simulink subsystem "HydrostaticCVT"  (R2025a)
settings: Solver=VariableStepAuto  StartTime=0.0  StopTime=10.0  RelTol=1e-3
undefined symbols (not defined in the file): fluids, hydrostaticCVT
libraries: fl_lib x48, nesl_utility x21, SimscapeFluids_lib x10
(part 1 of 2)
settings Model: Creator=varora  LastModifiedBy=varora

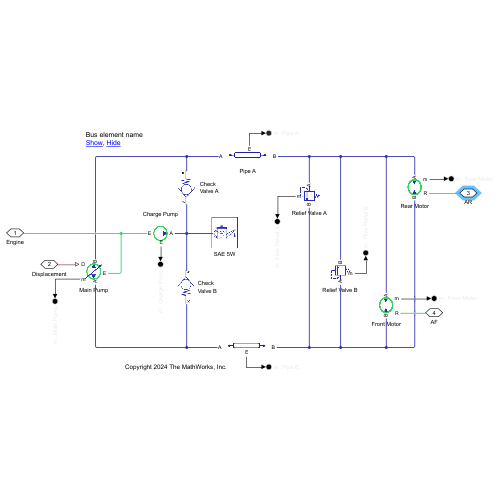
[thumbnail: Simulink's stored preview of the top-level diagram]
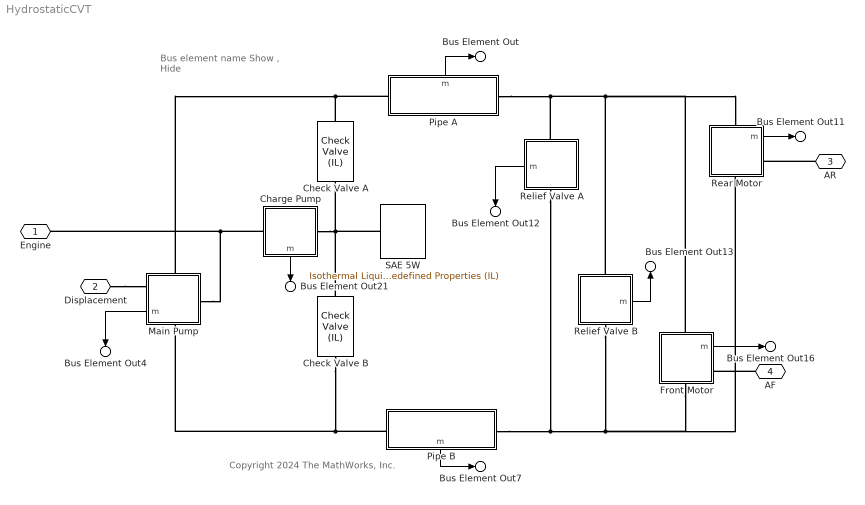
== system HydrostaticCVT ==
  note: Copyright 2024 The MathWorks, Inc.
  note: Bus element name
      | Show , Hide
  Charge Pump : Subsystem
      settings: PortSchema="{\"entries\":[{\"content\":{\"sides\":[{\"content\":{\"connectorIds\":[\"LConn1\"]},\"type\":\"ConnectorPlacement.EquallySpacedRectSide\",\"uuid\":\"81990219-23ac-4389-a887-166c20c53a41\"},{\"content\":{\"connectorIds\":[\"RConn1\"],\"side\":\"RIGHT\"},\"type\":\"ConnectorPlacement.EquallySpacedRectSide\",\"uuid\":\"3a415587-1da3-4934-b76c-e991c85e941a\"},{\"content\":{\"side\":\"TOP\"},\"type\":\"ConnectorPlacement.EquallySpacedRectSide\",\"uuid\":\"72b315a4-6c20-47a4-988f-efee67fcb81b\"},{\"content\":{\"connectorIds\":[\"Out1\"],\"side\":\"BOTTOM\"},\"type\":\"ConnectorPlacement.EquallySpacedRectSide\",\"uuid\":\"18a5ef52-f25e-4c35-ac51-885ef06c2aba\"}]},\"type\":\"ConnectorPlacement.EquallySpacedConnector\",\"uuid\":\"73b5088a-800b-40b1-b457-59a8e6f658c4\"}],\"packageUris\":[\"http://schema.mathworks.com/mf0/Connector/R2020b\"],\"version\":\"1.0\"}"
      mask Display: image('Fixed Displacement Pump.png');
  Check Valve A : SimscapeFluids_lib/Isothermal Liquid/Valves & Orifices/Directional Control Valves/Check Valve (IL)  opening_spec=2*(fluids.isothermal_liquid.valves_orifices.enum.PressureOpeningSpec.Linear)-1  pressure_control_spec=fluids.isothermal_liquid.valves_orifices.enum.pressure_control_spec.dp  p_crack_differential=hydrostaticCVT.pressDifferentialCracking MPa  p_crack_gauge=0.1 MPa  press_max_differential="hydrostaticCVT.pressDifferentialMaxOpen   MPa"  press_max_gauge=0.2 MPa  area_max=hydrostaticCVT.areaMax m^2  area_leak=hydrostaticCVT.areaLeak m^2  p_diff_TLU=[0.01 : 0.01 : 0.1] MPa  valve_area_TLU=[1e-10, 1e-05, 2e-05, 3e-05, 4e-05, 5e-05, 6e-05, 7.5e-05, 8.5e-05, .0001] m^2  vol_flow_TLU=[.000358, .045, .11, .191, .284, .39, .505, .63, .764, .905] .* 1e-3 m^3/s  area=inf m^2  Cd=hydrostaticCVT.cd  Re_c=150  smoothing_factor=0.01  pressure_recovery=simscape.enum.onoff.off  opening_dynamics=simscape.enum.onoff.off  tau=0.1 s
      settings: InternalSimscapePortConfiguration="{\"Bottom\":[],\"Left\":[{\"id\":\"A\",\"label\":\"A\",\"type\":\"foundation.isothermal_liquid.isothermal_liquid\"}],\"Right\":[{\"id\":\"B\",\"label\":\"B\",\"type\":\"foundation.isothermal_liquid.isothermal_liquid\"}],\"Top\":[]}"
  Check Valve B : SimscapeFluids_lib/Isothermal Liquid/Valves & Orifices/Directional Control Valves/Check Valve (IL)  opening_spec=2*(fluids.isothermal_liquid.valves_orifices.enum.PressureOpeningSpec.Linear)-1  pressure_control_spec=fluids.isothermal_liquid.valves_orifices.enum.pressure_control_spec.dp  p_crack_differential=hydrostaticCVT.pressDifferentialCracking MPa  p_crack_gauge=0.1 MPa  press_max_differential="hydrostaticCVT.pressDifferentialMaxOpen   MPa"  press_max_gauge=0.2 MPa  area_max=hydrostaticCVT.areaMax m^2  area_leak=hydrostaticCVT.areaLeak m^2  p_diff_TLU=[0.01 : 0.01 : 0.1] MPa  valve_area_TLU=[1e-10, 1e-05, 2e-05, 3e-05, 4e-05, 5e-05, 6e-05, 7.5e-05, 8.5e-05, .0001] m^2  vol_flow_TLU=[.000358, .045, .11, .191, .284, .39, .505, .63, .764, .905] .* 1e-3 m^3/s  area=inf m^2  Cd=hydrostaticCVT.cd  Re_c=150  smoothing_factor=0.01  pressure_recovery=simscape.enum.onoff.off  opening_dynamics=simscape.enum.onoff.off  tau=0.1 s
      settings: InternalSimscapePortConfiguration="{\"Bottom\":[],\"Left\":[{\"id\":\"A\",\"label\":\"A\",\"type\":\"foundation.isothermal_liquid.isothermal_liquid\"}],\"Right\":[{\"id\":\"B\",\"label\":\"B\",\"type\":\"foundation.isothermal_liquid.isothermal_liquid\"}],\"Top\":[]}"
  Front Motor : Subsystem
      settings: PortSchema="{\"entries\":[{\"content\":{\"sides\":[{\"content\":{},\"type\":\"ConnectorPlacement.EquallySpacedRectSide\",\"uuid\":\"af94f2aa-b04e-40af-a187-0818155794dd\"},{\"content\":{\"connectorIds\":[\"Out1\",\"RConn1\"],\"side\":\"RIGHT\"},\"type\":\"ConnectorPlacement.EquallySpacedRectSide\",\"uuid\":\"5c20c2e1-8527-47fe-9ffe-16d60e314a5b\"},{\"content\":{\"connectorIds\":[\"LConn1\"],\"side\":\"TOP\"},\"type\":\"ConnectorPlacement.EquallySpacedRectSide\",\"uuid\":\"e7f5e70d-3df0-46cd-83a4-29ec656a12c9\"},{\"content\":{\"connectorIds\":[\"RConn2\"],\"side\":\"BOTTOM\"},\"type\":\"ConnectorPlacement.EquallySpacedRectSide\",\"uuid\":\"f2252cf3-f3a6-42d9-8396-2baa411525c5\"}]},\"type\":\"ConnectorPlacement.EquallySpacedConnector\",\"uuid\":\"0c7ba87d-5f8c-4429-8766-c6dc02a36f7b\"}],\"packageUris\":[\"http://schema.mathworks.com/mf0/Connector/R2020b\"],\"version\":\"1.0\"}"
      mask Display: image('Fixed Displacement Motor.png');
  Main Pump : Subsystem
      settings: PortSchema="{\"entries\":[{\"content\":{\"sides\":[{\"content\":{\"connectorIds\":[\"LConn1\",\"Out1\"]},\"type\":\"ConnectorPlacement.EquallySpacedRectSide\",\"uuid\":\"857969f3-473a-4560-b879-851e5f4c83b0\"},{\"content\":{\"connectorIds\":[\"RConn1\"],\"side\":\"RIGHT\"},\"type\":\"ConnectorPlacement.EquallySpacedRectSide\",\"uuid\":\"4f69d4a9-a494-47de-b36f-c1227f8f36db\"},{\"content\":{\"connectorIds\":[\"LConn2\"],\"side\":\"TOP\"},\"type\":\"ConnectorPlacement.EquallySpacedRectSide\",\"uuid\":\"5719fdc2-cb8a-4698-a7b4-0c22c79051ee\"},{\"content\":{\"connectorIds\":[\"RConn2\"],\"side\":\"BOTTOM\"},\"type\":\"ConnectorPlacement.EquallySpacedRectSide\",\"uuid\":\"9c51d1b2-abf1-46a3-9cf9-9060aeca44d8\"}]},\"type\":\"ConnectorPlacement.EquallySpacedConnector\",\"uuid\":\"aaa09012-c93e-45df-8a88-38540d88c81c\"}],\"packageUris\":[\"http://schema.mathworks.com/mf0/Connector/R2020b\"],\"version\":\"1.0\"}"
      mask Display: image('Variable Displacement Pump.png');
  Pipe A : Subsystem
      settings: PortSchema="{\"entries\":[{\"content\":{\"sides\":[{\"content\":{\"connectorIds\":[\"LConn1\"]},\"type\":\"ConnectorPlacement.EquallySpacedRectSide\",\"uuid\":\"d71b6971-6f33-4ff5-9472-1e7ceb29be5c\"},{\"content\":{\"connectorIds\":[\"RConn1\"],\"side\":\"RIGHT\"},\"type\":\"ConnectorPlacement.EquallySpacedRectSide\",\"uuid\":\"20efd35b-04f1-44a0-a5ae-b6ecc8cce91a\"},{\"content\":{\"connectorIds\":[\"Out1\"],\"side\":\"TOP\"},\"type\":\"ConnectorPlacement.EquallySpacedRectSide\",\"uuid\":\"941ffbf3-e51b-4589-ab00-835957186b5f\"}]},\"type\":\"ConnectorPlacement.EquallySpacedConnector\",\"uuid\":\"7b30b026-434b-4245-94a4-5fd456974538\"}],\"packageUris\":[\"http://schema.mathworks.com/mf0/Connector/R2020b\"],\"version\":\"1.0\"}"
      mask Display: image('Pipe.png');
  Pipe B : Subsystem
      settings: PortSchema="{\"entries\":[{\"content\":{\"sides\":[{\"content\":{\"connectorIds\":[\"LConn1\"]},\"type\":\"ConnectorPlacement.EquallySpacedRectSide\",\"uuid\":\"d71b6971-6f33-4ff5-9472-1e7ceb29be5c\"},{\"content\":{\"connectorIds\":[\"RConn1\"],\"side\":\"RIGHT\"},\"type\":\"ConnectorPlacement.EquallySpacedRectSide\",\"uuid\":\"20efd35b-04f1-44a0-a5ae-b6ecc8cce91a\"},{\"content\":{\"side\":\"TOP\"},\"type\":\"ConnectorPlacement.EquallySpacedRectSide\",\"uuid\":\"941ffbf3-e51b-4589-ab00-835957186b5f\"},{\"content\":{\"connectorIds\":[\"Out1\"],\"side\":\"BOTTOM\"},\"type\":\"ConnectorPlacement.EquallySpacedRectSide\",\"uuid\":\"a318eed9-4e9d-48d8-b72b-a2a7d74f41ab\"}]},\"type\":\"ConnectorPlacement.EquallySpacedConnector\",\"uuid\":\"7b30b026-434b-4245-94a4-5fd456974538\"}],\"packageUris\":[\"http://schema.mathworks.com/mf0/Connector/R2020b\"],\"version\":\"1.0\"}"
      mask Display: image('Pipe.png');
  Rear Motor : Subsystem
      settings: PortSchema="{\"entries\":[{\"content\":{\"sides\":[{\"content\":{},\"type\":\"ConnectorPlacement.EquallySpacedRectSide\",\"uuid\":\"af94f2aa-b04e-40af-a187-0818155794dd\"},{\"content\":{\"connectorIds\":[\"Out1\",\"RConn1\"],\"side\":\"RIGHT\"},\"type\":\"ConnectorPlacement.EquallySpacedRectSide\",\"uuid\":\"5c20c2e1-8527-47fe-9ffe-16d60e314a5b\"},{\"content\":{\"connectorIds\":[\"LConn1\"],\"side\":\"TOP\"},\"type\":\"ConnectorPlacement.EquallySpacedRectSide\",\"uuid\":\"e7f5e70d-3df0-46cd-83a4-29ec656a12c9\"},{\"content\":{\"connectorIds\":[\"RConn2\"],\"side\":\"BOTTOM\"},\"type\":\"ConnectorPlacement.EquallySpacedRectSide\",\"uuid\":\"960debcf-3e01-48e5-86cf-b4bb7f8de203\"}]},\"type\":\"ConnectorPlacement.EquallySpacedConnector\",\"uuid\":\"0c7ba87d-5f8c-4429-8766-c6dc02a36f7b\"}],\"packageUris\":[\"http://schema.mathworks.com/mf0/Connector/R2020b\"],\"version\":\"1.0\"}"
      mask Display: image('Fixed Displacement Motor.png');
  Relief Valve A : Subsystem
      settings: PortSchema="{\"entries\":[{\"content\":{\"sides\":[{\"content\":{\"connectorIds\":[\"LConn1\"]},\"type\":\"ConnectorPlacement.EquallySpacedRectSide\",\"uuid\":\"a381c46d-7477-4f99-8d1a-7d1a868f6356\"},{\"content\":{\"connectorIds\":[\"RConn1\"],\"side\":\"RIGHT\"},\"type\":\"ConnectorPlacement.EquallySpacedRectSide\",\"uuid\":\"1773284f-5c53-4cb3-9146-19bcc89e0bf2\"},{\"content\":{\"connectorIds\":[\"Out1\"],\"side\":\"TOP\"},\"type\":\"ConnectorPlacement.EquallySpacedRectSide\",\"uuid\":\"2cc97cf0-3f11-430a-9e32-d4b384bcc7e2\"}]},\"type\":\"ConnectorPlacement.EquallySpacedConnector\",\"uuid\":\"a3df120c-9f95-4600-8cbc-77d57dad487f\"}],\"packageUris\":[\"http://schema.mathworks.com/mf0/Connector/R2020b\"],\"version\":\"1.0\"}"
      mask Display: image('Relief Valve.png');
  Relief Valve B : Subsystem
      settings: PortSchema="{\"entries\":[{\"content\":{\"sides\":[{\"content\":{\"connectorIds\":[\"LConn1\"]},\"type\":\"ConnectorPlacement.EquallySpacedRectSide\",\"uuid\":\"a381c46d-7477-4f99-8d1a-7d1a868f6356\"},{\"content\":{\"connectorIds\":[\"RConn1\"],\"side\":\"RIGHT\"},\"type\":\"ConnectorPlacement.EquallySpacedRectSide\",\"uuid\":\"1773284f-5c53-4cb3-9146-19bcc89e0bf2\"},{\"content\":{\"side\":\"TOP\"},\"type\":\"ConnectorPlacement.EquallySpacedRectSide\",\"uuid\":\"2cc97cf0-3f11-430a-9e32-d4b384bcc7e2\"},{\"content\":{\"connectorIds\":[\"Out1\"],\"side\":\"BOTTOM\"},\"type\":\"ConnectorPlacement.EquallySpacedRectSide\",\"uuid\":\"486595bc-126c-4ff1-8e4a-4a4a030a425b\"}]},\"type\":\"ConnectorPlacement.EquallySpacedConnector\",\"uuid\":\"a3df120c-9f95-4600-8cbc-77d57dad487f\"}],\"packageUris\":[\"http://schema.mathworks.com/mf0/Connector/R2020b\"],\"version\":\"1.0\"}"
      mask Display: image('Relief Valve.png');
  SAE 5W : SimscapeFluids_lib/Isothermal Liquid/Utilities/Isothermal Liquid Predefined Properties (IL)  fluid_list=fluids.isothermal_liquid.utilities.enum.isothermal_liquid_fluid_list.sae5w30  concentration_param_EG=fluids.isothermal_liquid.utilities.enum.isothermal_liquid_concentration.volume_fraction  concentration_param_PG=fluids.isothermal_liquid.utilities.enum.isothermal_liquid_concentration.volume_fraction  c_mass_SW=3.5e-3  c_mass_EG=0.1  c_mass_PG=0.1  c_mass_GL=0.1  c_vol_EG=0.1  c_vol_PG=0.1  beta_L_atm_EG=2.1791 GPa  beta_L_atm_PG=2.1791 GPa  beta_L_atm_GL=2.1791 GPa  p_min_EG=0.01 MPa  p_min_PG=0.01 MPa  p_min_GL=0.01 MPa  T=293.15 K  derate_coeff=1  p_atm=0.101325 MPa  properties_range_check=simscape.enum.assert.action.error  air_fraction=0.02  polytropic_index=1.0  rho_g_atm=1.225 kg/m^3  air_dissolution_model=simscape.enum.onoff.off  p_crit=3 MPa
      settings: InternalSimscapePortConfiguration="{\"Bottom\":[],\"Left\":[],\"Right\":[{\"id\":\"A\",\"label\":\"\",\"type\":\"foundation.isothermal_liquid.isothermal_liquid\"}],\"Top\":[]}"
  Engine : PMIOPort  Side=Left
  Displacement : PMIOPort  Port=2  Side=Left
  AR : PMIOPort  Port=3  Side=Right
  AF : PMIOPort  Port=4  Side=Right
  Bus Element Out : Outport  PortName=m  Element=Pipe A
  Bus Element Out4 : Outport  PortName=m  Element=Main Pump
  Bus Element Out7 : Outport  PortName=m  Element=Pipe B
  Bus Element Out11 : Outport  PortName=m  Element=Rear Motor
  Bus Element Out12 : Outport  PortName=m  Element=Flow Relief A
  Bus Element Out13 : Outport  PortName=m  Element=Flow Relief B
  Bus Element Out16 : Outport  PortName=m  Element=Front Motor
  Bus Element Out21 : Outport  PortName=m  Element=Charge Pump
  wires:
  Main Pump/1(m) -> Bus Element Out4/1
  Pipe A/1(m) -> Bus Element Out/1
  Pipe B/1(m) -> Bus Element Out7/1
  Front Motor/1(m) -> Bus Element Out16/1
  Rear Motor/1(m) -> Bus Element Out11/1
  Relief Valve A/1(m) -> Bus Element Out12/1
  Relief Valve B/1(m) -> Bus Element Out13/1
  Charge Pump/1(m) -> Bus Element Out21/1
  connections:
  Main Pump/LConn2 -- Pipe A/LConn1 -- Check Valve A/RConn1
  SAE 5W/RConn1 -- Charge Pump/RConn1 -- Check Valve B/LConn1 -- Check Valve A/LConn1
  Pipe A/RConn1 -- Rear Motor/LConn1 -- Front Motor/LConn1 -- Relief Valve B/RConn1 -- Relief Valve A/LConn1
  Pipe B/LConn1 -- Check Valve B/RConn1 -- Main Pump/RConn2
  Pipe B/RConn1 -- Rear Motor/RConn2 -- Front Motor/RConn2 -- Relief Valve B/LConn1 -- Relief Valve A/RConn1
  Main Pump/RConn1 -- Charge Pump/LConn1 -- Engine/RConn1
  Displacement/RConn1 -- Main Pump/LConn1
  AF/RConn1 -- Front Motor/RConn1
  AR/RConn1 -- Rear Motor/RConn1

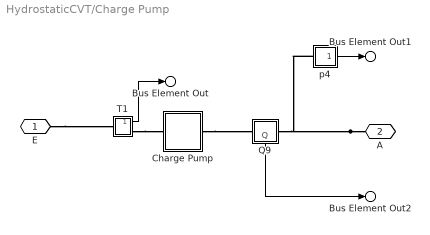
== system HydrostaticCVT/Charge Pump ==
  Charge Pump : Subsystem  Tag=PublishSubsystem
      mask Display:
      | % Circle
      | plot(2*cos(linspace(0, 2*pi, 100)), 2*sin(linspace(0, 2*pi, 100)))
      | % Triangle
      | patch([1 0.4 0.4]*2, [0,-0.4,0.4]*2)
      | % Boundary
      | color('white')
      | plot(-2, -2)
      | plot(2, 2)
  Q9 : Subsystem
      settings: PortSchema="{\"entries\":[{\"content\":{\"sides\":[{\"content\":{},\"type\":\"ConnectorPlacement.EquallySpacedRectSide\",\"uuid\":\"a381c46d-7477-4f99-8d1a-7d1a868f6356\"},{\"content\":{\"connectorIds\":[\"Out1\"],\"side\":\"RIGHT\"},\"type\":\"ConnectorPlacement.EquallySpacedRectSide\",\"uuid\":\"1773284f-5c53-4cb3-9146-19bcc89e0bf2\"},{\"content\":{\"connectorIds\":[\"LConn1\"],\"side\":\"TOP\"},\"type\":\"ConnectorPlacement.EquallySpacedRectSide\",\"uuid\":\"2cc97cf0-3f11-430a-9e32-d4b384bcc7e2\"},{\"content\":{\"connectorIds\":[\"RConn1\"],\"side\":\"BOTTOM\"},\"type\":\"ConnectorPlacement.EquallySpacedRectSide\",\"uuid\":\"6b1044f7-a51c-47fb-9697-f1e3b42da025\"}]},\"type\":\"ConnectorPlacement.EquallySpacedConnector\",\"uuid\":\"a3df120c-9f95-4600-8cbc-77d57dad487f\"}],\"packageUris\":[\"http://schema.mathworks.com/mf0/Connector/R2020b\"],\"version\":\"1.0\"}"
      mask Display: disp('Q')
  T1 : Subsystem
      mask Display: disp('S')
  p4 : Subsystem
      mask Display: disp('P')
  E : PMIOPort  Side=Left
  A : PMIOPort  Port=2  Side=Right
  Bus Element Out : Outport  PortName=m  Element=trq (N*m)
  Bus Element Out1 : Outport  PortName=m  Element=P (bar)
  Bus Element Out2 : Outport  PortName=m  Element=q (m^3/s)
  wires:
  Q9/1(Q) -> Bus Element Out2/1
  p4/1(" P") -> Bus Element Out1/1
  T1/1(T) -> Bus Element Out/1
  connections:
  T1/RConn1 -- Charge Pump/LConn1
  Charge Pump/RConn1 -- Q9/RConn1
  E/RConn1 -- T1/LConn1
  A/RConn1 -- Q9/LConn1 -- p4/LConn1

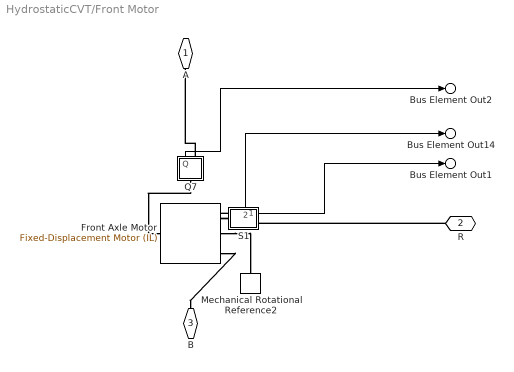
== system HydrostaticCVT/Front Motor ==
  Front Axle Motor : SimscapeFluids_lib/Isothermal Liquid/Pumps & Motors/Fixed-Displacement Motor (IL)  leakage_friction_spec=fluids.isothermal_liquid.pumps_motors.enum.MotorLossSpec.Analytical  displacement=hydrostaticCVT.displacementMotor cm^3/rev  omega_nominal=hydrostaticCVT.shaftVelocityNominal rpm  p_nominal=hydrostaticCVT.nominalPressureGain MPa  vol_eff_nominal=hydrostaticCVT.efficiencyVolumetric  mech_eff_nominal=hydrostaticCVT.efficiencyMechanical  no_load_torque=0 N*m  p_diff_eff_TLU=[.1, 1, 2] MPa  omega_eff_TLU=[25, 50, 100, 200, 300, 400] rad/s  vol_eff_TLU=[.816, .908, .954, .977, .981, .984; .325, .663, .831, .916, .925, .946; .137, .568, .78, .892, .893, .91]  mech_eff_TLU=[.996, .996, .996, .996, .996, .996; .988, .989, .989, .989, .989, .99; .981, .981, .982, .982, .983, .984]  p_diff_loss_TLU=[.1, 1, 2] MPa  omega_loss_TLU=[25, 50, 100, 200, 300, 400] rad/s  vol_loss_TLU=[.023, .023, .023, .023, .0285, .032; .0844, .0842, .0845, .084, .1125, .108; .1079, .108, .11, .108, .1605, .18] * 1e-3 m^3/s  mech_loss_TLU=[.002, .002, .002, .002, .002, .002; .0607, .0556, .0556, .0556, .0556, .0505; .1937, .1937, .1833, .1833, .1729, .1626] N*m  q_shaft_TLU=[.125, .25, .5, 1, 1.5, 2] * 1e-3 m^3/s  p_diff_shaft_TLU=[.1, 1, 2] MPa  torque_shaft_TLU=[.47, 4.72, 9.35; .47, 4.7, 9.36; .47, 4.7, 9.4; .47, 4.7, 9.41; .47, 4.7, 9.46; .47, 4.68, 9.5] N*m  omega_shaft_TLU=[205, 80, 35; 455, 330, 285; 955, 831, 780; 1950, 1830, 1780; 2940, 2775, 2680; 3940, 3780, 3640] rpm  vol_eff_min=1e-3  vol_eff_max=1  mech_eff_min=1e-3  mech_eff_max=1  pressure_threshold=1e-3 MPa  omega_threshold=10 rad/s  supplied_range_check=simscape.enum.assert.action.none  motor_mode_check=simscape.enum.assert.action.none  pressure_check=simscape.enum.assert.action.none  p_min_valid=0.101325 MPa
      settings: InternalSimscapePortConfiguration="{\"Bottom\":[{\"id\":\"B\",\"label\":\"B\",\"type\":\"foundation.isothermal_liquid.isothermal_liquid\"}],\"Left\":[],\"Right\":[{\"id\":\"R\",\"label\":\"R\",\"type\":\"foundation.mechanical.rotational.rotational\"},{\"id\":\"C\",\"label\":\"C\",\"type\":\"foundation.mechanical.rotational.rotational\"}],\"Top\":[{\"id\":\"A\",\"label\":\"A\",\"type\":\"foundation.isothermal_liquid.isothermal_liquid\"}]}"
  Mechanical Rotational Reference2 : fl_lib/Mechanical/Rotational Elements/Mechanical Rotational Reference
  Q7 : Subsystem
      mask Display: disp('Q')
  S1 : Subsystem
      settings: PortSchema="{\"entries\":[{\"content\":{\"sides\":[{\"content\":{\"connectorIds\":[\"LConn1\"]},\"type\":\"ConnectorPlacement.EquallySpacedRectSide\",\"uuid\":\"d71b6971-6f33-4ff5-9472-1e7ceb29be5c\"},{\"content\":{\"connectorIds\":[\"Out1\",\"RConn1\"],\"side\":\"RIGHT\"},\"type\":\"ConnectorPlacement.EquallySpacedRectSide\",\"uuid\":\"20efd35b-04f1-44a0-a5ae-b6ecc8cce91a\"},{\"content\":{\"connectorIds\":[\"Out2\"],\"side\":\"TOP\"},\"type\":\"ConnectorPlacement.EquallySpacedRectSide\",\"uuid\":\"941ffbf3-e51b-4589-ab00-835957186b5f\"}]},\"type\":\"ConnectorPlacement.EquallySpacedConnector\",\"uuid\":\"7b30b026-434b-4245-94a4-5fd456974538\"}],\"packageUris\":[\"http://schema.mathworks.com/mf0/Connector/R2020b\"],\"version\":\"1.0\"}"
      mask Display: disp('S')
  A : PMIOPort  Side=Left
  R : PMIOPort  Port=2  Side=Right
  B : PMIOPort  Port=3  Side=Right
  Bus Element Out14 : Outport  PortName=m  Element=w (rpm)
  Bus Element Out1 : Outport  PortName=m  Element=trq (N*m)
  Bus Element Out2 : Outport  PortName=m  Element=q (m^3/s)
  wires:
  Q7/1(Q) -> Bus Element Out2/1
  S1/1(T (N*m)) -> Bus Element Out1/1
  S1/2(w (rpm)) -> Bus Element Out14/1
  connections:
  Q7/RConn1 -- A/RConn1
  Front Axle Motor/RConn3 -- B/RConn1
  Front Axle Motor/RConn2 -- Mechanical Rotational Reference2/LConn1
  R/RConn1 -- S1/RConn1
  Q7/LConn1 -- Front Axle Motor/LConn1
  S1/LConn1 -- Front Axle Motor/RConn1

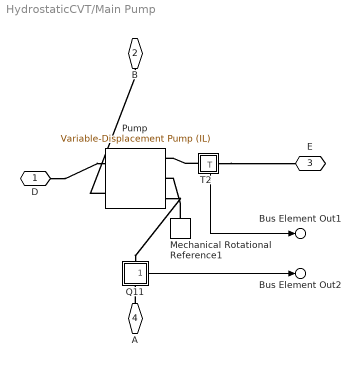
== system HydrostaticCVT/Main Pump ==
  Mechanical Rotational Reference1 : fl_lib/Mechanical/Rotational Elements/Mechanical Rotational Reference
  Pump : SimscapeFluids_lib/Isothermal Liquid/Pumps & Motors/Variable-Displacement Pump (IL)  leakage_friction_spec=fluids.isothermal_liquid.pumps_motors.enum.pump_motor_loss_spec.analytical  displacement_nominal=hydrostaticCVT.displacementPump cm^3/rev  omega_nominal=hydrostaticCVT.shaftVelocityNominal rpm  p_nominal=hydrostaticCVT.nominalPressureGain MPa  vol_eff_nominal=hydrostaticCVT.efficiencyVolumetric  mech_eff_nominal=hydrostaticCVT.efficiencyMechanical  no_load_torque=0 N*m  p_diff_eff_TLU=[.1, 1, 2] MPa  omega_eff_TLU=[25, 50, 100, 200, 300, 400] rad/s  displacement_eff_TLU=[-30, -19, 19, 30] cm^3/rev  vol_eff_TLU=repmat([.816, .908, .954, .977, .981, .984; .325, .663, .831, .916, .925, .946; .137, .568, .78, .892, .893, .91], 1, 1, 4)  mech_eff_TLU=repmat([.996, .996, .996, .996, .996, .996; .988, .989, .989, .989, .989, .99; .981, .981, .982, .982, .983, .984], 1, 1, 4)  p_diff_loss_TLU=[.1, 1, 2] MPa  omega_loss_TLU=[25, 50, 100, 200, 300, 400] rad/s  displacement_loss_TLU=[-30, -19, 19, 30] cm^3/rev  vol_loss_TLU=repmat([.023, .023, .023, .023, .0285, .032; .0844, .0842, .0845, .084, .1125, .108; .1079, .108, .11, .108, .1605, .18] * 1e-3, 1, 1, 4) m^3/s  mech_loss_TLU=repmat([.002, .002, .002, .002, .002, .002; .0607, .0556, .0556, .0556, .0556, .0505; .1937, .1937, .1833, .1833, .1729, .1626], 1, 1, 4) N*m  vol_eff_min=1e-3  vol_eff_max=1  mech_eff_min=1e-3  mech_eff_max=1  pressure_threshold=1e-3 MPa  omega_threshold=10 rad/s  displacement_threshold=0.1 cm^3/rev  supplied_range_check=simscape.enum.assert.action.none  pump_mode_check=simscape.enum.assert.action.none  pressure_check=simscape.enum.assert.action.none  p_min_valid=0.101325 MPa
      settings: InternalSimscapePortConfiguration="{\"Bottom\":[{\"id\":\"A\",\"label\":\"A\",\"type\":\"foundation.isothermal_liquid.isothermal_liquid\"}],\"Left\":[{\"id\":\"D\",\"label\":\"D\",\"type\":\"input\"}],\"Right\":[{\"id\":\"R\",\"label\":\"R\",\"type\":\"foundation.mechanical.rotational.rotational\"},{\"id\":\"C\",\"label\":\"C\",\"type\":\"foundation.mechanical.rotational.rotational\"}],\"Top\":[{\"id\":\"B\",\"label\":\"B\",\"type\":\"foundation.isothermal_liquid.isothermal_liquid\"}]}"
  Q11 : Subsystem
      settings: PortSchema="{\"entries\":[{\"content\":{\"sides\":[{\"content\":{\"connectorIds\":[\"LConn1\"]},\"type\":\"ConnectorPlacement.EquallySpacedRectSide\",\"uuid\":\"a381c46d-7477-4f99-8d1a-7d1a868f6356\"},{\"content\":{\"connectorIds\":[\"RConn1\"],\"side\":\"RIGHT\"},\"type\":\"ConnectorPlacement.EquallySpacedRectSide\",\"uuid\":\"1773284f-5c53-4cb3-9146-19bcc89e0bf2\"},{\"content\":{\"side\":\"TOP\"},\"type\":\"ConnectorPlacement.EquallySpacedRectSide\",\"uuid\":\"2cc97cf0-3f11-430a-9e32-d4b384bcc7e2\"},{\"content\":{\"connectorIds\":[\"Out1\"],\"side\":\"BOTTOM\"},\"type\":\"ConnectorPlacement.EquallySpacedRectSide\",\"uuid\":\"73fb13f1-32e6-4f88-8a39-50ddc70c8cb7\"}]},\"type\":\"ConnectorPlacement.EquallySpacedConnector\",\"uuid\":\"a3df120c-9f95-4600-8cbc-77d57dad487f\"}],\"packageUris\":[\"http://schema.mathworks.com/mf0/Connector/R2020b\"],\"version\":\"1.0\"}"
      mask Display: disp('Q')
  T2 : Subsystem
      settings: PortSchema="{\"entries\":[{\"content\":{\"sides\":[{\"content\":{\"connectorIds\":[\"LConn1\"]},\"type\":\"ConnectorPlacement.EquallySpacedRectSide\",\"uuid\":\"a381c46d-7477-4f99-8d1a-7d1a868f6356\"},{\"content\":{\"connectorIds\":[\"RConn1\"],\"side\":\"RIGHT\"},\"type\":\"ConnectorPlacement.EquallySpacedRectSide\",\"uuid\":\"1773284f-5c53-4cb3-9146-19bcc89e0bf2\"},{\"content\":{\"side\":\"TOP\"},\"type\":\"ConnectorPlacement.EquallySpacedRectSide\",\"uuid\":\"2cc97cf0-3f11-430a-9e32-d4b384bcc7e2\"},{\"content\":{\"connectorIds\":[\"Out1\"],\"side\":\"BOTTOM\"},\"type\":\"ConnectorPlacement.EquallySpacedRectSide\",\"uuid\":\"68438fb6-2ad6-4198-8251-4c01567bf9f2\"}]},\"type\":\"ConnectorPlacement.EquallySpacedConnector\",\"uuid\":\"a3df120c-9f95-4600-8cbc-77d57dad487f\"}],\"packageUris\":[\"http://schema.mathworks.com/mf0/Connector/R2020b\"],\"version\":\"1.0\"}"
      mask Display: disp('S')
  D : PMIOPort  Side=Left
  B : PMIOPort  Port=2  Side=Left
  E : PMIOPort  Port=3  Side=Right
  A : PMIOPort  Port=4  Side=Right
  Bus Element Out1 : Outport  PortName=m  Element=trq (N*m)
  Bus Element Out2 : Outport  PortName=m  Element=q (m^3/s)
  wires:
  Q11/1(Q) -> Bus Element Out2/1
  T2/1(T) -> Bus Element Out1/1
  connections:
  A/RConn1 -- Q11/LConn1
  Pump/RConn3 -- Q11/RConn1
  Pump/LConn2 -- B/RConn1
  D/RConn1 -- Pump/LConn1
  T2/LConn1 -- E/RConn1
  Mechanical Rotational Reference1/LConn1 -- Pump/RConn2
  T2/RConn1 -- Pump/RConn1

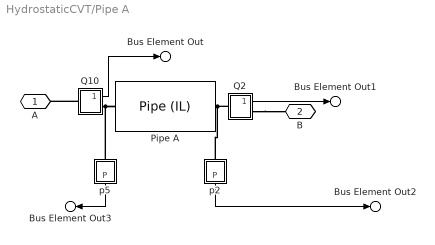
== system HydrostaticCVT/Pipe A ==
  Pipe A : fl_lib/Isothermal Liquid/Elements/Pipe (IL)  length=hydrostaticCVT.lengthPipe m  area=pi * hydrostaticCVT.diameterPipe^2 / 4 m^2  Dh=hydrostaticCVT.diameterPipe m  length_add=hydrostaticCVT.lengthPipe*0.5 m  roughness=30e-6 m  Re_lam=2000  Re_tur=4000  shape_factor=64  dynamic_compressibility=simscape.enum.onoff.on  inertia=simscape.enum.onoff.off  p0=0.101325 MPa  mdot0=0 kg/s
      settings: InternalSimscapePortConfiguration="{\"Bottom\":[],\"Left\":[{\"id\":\"A\",\"label\":\"A\",\"type\":\"foundation.isothermal_liquid.isothermal_liquid\"}],\"Right\":[{\"id\":\"B\",\"label\":\"B\",\"type\":\"foundation.isothermal_liquid.isothermal_liquid\"}],\"Top\":[]}"
  Q10 : Subsystem
      mask Display: disp('Q')
  Q2 : Subsystem
      mask Display: disp('Q')
  p2 : Subsystem
      mask Display: disp('P')
  p5 : Subsystem
      mask Display: disp('P')
  A : PMIOPort  Side=Left
  B : PMIOPort  Port=2  Side=Right
  Bus Element Out : Outport  PortName=m  Element=qA (m^3/s)
  Bus Element Out1 : Outport  PortName=m  Element=qB (m^3/s)
  Bus Element Out2 : Outport  PortName=m  Element=pB (bar)
  Bus Element Out3 : Outport  PortName=m  Element=pA (bar)
  wires:
  p5/1(" P") -> Bus Element Out3/1
  p2/1(" P") -> Bus Element Out2/1
  Q2/1(Q) -> Bus Element Out1/1
  Q10/1(Q) -> Bus Element Out/1
  connections:
  Q2/RConn1 -- B/RConn1
  Q10/LConn1 -- A/RConn1
  p2/LConn1 -- Q2/LConn1 -- Pipe A/RConn1
  p5/LConn1 -- Pipe A/LConn1 -- Q10/RConn1

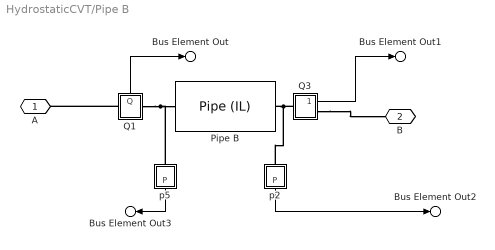
== system HydrostaticCVT/Pipe B ==
  Pipe B : fl_lib/Isothermal Liquid/Elements/Pipe (IL)  length=hydrostaticCVT.lengthPipe m  area=pi * hydrostaticCVT.diameterPipe^2 / 4 m^2  Dh=hydrostaticCVT.diameterPipe m  length_add=hydrostaticCVT.lengthPipe*0.5 m  roughness=30e-6 m  Re_lam=2000  Re_tur=4000  shape_factor=64  dynamic_compressibility=simscape.enum.onoff.on  inertia=simscape.enum.onoff.off  p0=0.101325 MPa  mdot0=0 kg/s
      settings: InternalSimscapePortConfiguration="{\"Bottom\":[],\"Left\":[{\"id\":\"A\",\"label\":\"A\",\"type\":\"foundation.isothermal_liquid.isothermal_liquid\"}],\"Right\":[{\"id\":\"B\",\"label\":\"B\",\"type\":\"foundation.isothermal_liquid.isothermal_liquid\"}],\"Top\":[]}"
  Q1 : Subsystem
      settings: PortSchema="{\"entries\":[{\"content\":{\"sides\":[{\"content\":{\"connectorIds\":[\"LConn1\"]},\"type\":\"ConnectorPlacement.EquallySpacedRectSide\",\"uuid\":\"a381c46d-7477-4f99-8d1a-7d1a868f6356\"},{\"content\":{\"connectorIds\":[\"RConn1\"],\"side\":\"RIGHT\"},\"type\":\"ConnectorPlacement.EquallySpacedRectSide\",\"uuid\":\"1773284f-5c53-4cb3-9146-19bcc89e0bf2\"},{\"content\":{\"side\":\"TOP\"},\"type\":\"ConnectorPlacement.EquallySpacedRectSide\",\"uuid\":\"2cc97cf0-3f11-430a-9e32-d4b384bcc7e2\"},{\"content\":{\"connectorIds\":[\"Out1\"],\"side\":\"BOTTOM\"},\"type\":\"ConnectorPlacement.EquallySpacedRectSide\",\"uuid\":\"9bce3d8d-32fe-4fbf-aee9-895eb85fad54\"}]},\"type\":\"ConnectorPlacement.EquallySpacedConnector\",\"uuid\":\"a3df120c-9f95-4600-8cbc-77d57dad487f\"}],\"packageUris\":[\"http://schema.mathworks.com/mf0/Connector/R2020b\"],\"version\":\"1.0\"}"
      mask Display: disp('Q')
  Q3 : Subsystem
      mask Display: disp('Q')
  p2 : Subsystem
      mask Display: disp('P')
  p5 : Subsystem
      mask Display: disp('P')
  A : PMIOPort  Side=Left
  B : PMIOPort  Port=2  Side=Right
  Bus Element Out : Outport  PortName=m  Element=qA (m^3/s)
  Bus Element Out1 : Outport  PortName=m  Element=qB (m^3/s)
  Bus Element Out2 : Outport  PortName=m  Element=pB (bar)
  Bus Element Out3 : Outport  PortName=m  Element=pA (bar)
  wires:
  Q1/1(Q) -> Bus Element Out/1
  p5/1(" P") -> Bus Element Out3/1
  Q3/1(Q) -> Bus Element Out1/1
  p2/1(" P") -> Bus Element Out2/1
  connections:
  Q1/LConn1 -- A/RConn1
  Q3/RConn1 -- B/RConn1
  p5/LConn1 -- Q1/RConn1 -- Pipe B/LConn1
  p2/LConn1 -- Q3/LConn1 -- Pipe B/RConn1

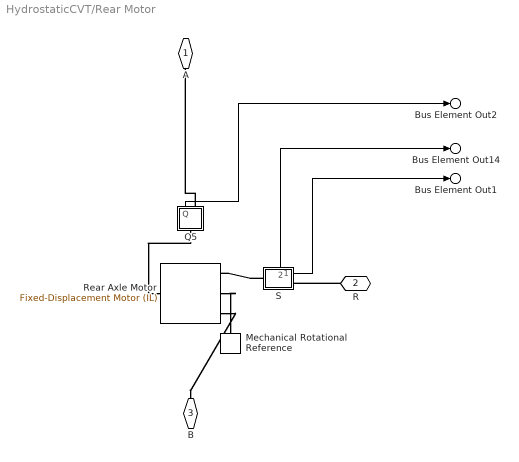
== system HydrostaticCVT/Rear Motor ==
  Mechanical Rotational Reference : fl_lib/Mechanical/Rotational Elements/Mechanical Rotational Reference
  Q5 : Subsystem
      mask Display: disp('Q')
  Rear Axle Motor : SimscapeFluids_lib/Isothermal Liquid/Pumps & Motors/Fixed-Displacement Motor (IL)  leakage_friction_spec=fluids.isothermal_liquid.pumps_motors.enum.MotorLossSpec.Analytical  displacement=hydrostaticCVT.displacementMotor cm^3/rev  omega_nominal=hydrostaticCVT.shaftVelocityNominal rpm  p_nominal=hydrostaticCVT.nominalPressureGain MPa  vol_eff_nominal=hydrostaticCVT.efficiencyVolumetric  mech_eff_nominal=hydrostaticCVT.efficiencyMechanical  no_load_torque=0 N*m  p_diff_eff_TLU=[.1, 1, 2] MPa  omega_eff_TLU=[25, 50, 100, 200, 300, 400] rad/s  vol_eff_TLU=[.816, .908, .954, .977, .981, .984; .325, .663, .831, .916, .925, .946; .137, .568, .78, .892, .893, .91]  mech_eff_TLU=[.996, .996, .996, .996, .996, .996; .988, .989, .989, .989, .989, .99; .981, .981, .982, .982, .983, .984]  p_diff_loss_TLU=[.1, 1, 2] MPa  omega_loss_TLU=[25, 50, 100, 200, 300, 400] rad/s  vol_loss_TLU=[.023, .023, .023, .023, .0285, .032; .0844, .0842, .0845, .084, .1125, .108; .1079, .108, .11, .108, .1605, .18] * 1e-3 m^3/s  mech_loss_TLU=[.002, .002, .002, .002, .002, .002; .0607, .0556, .0556, .0556, .0556, .0505; .1937, .1937, .1833, .1833, .1729, .1626] N*m  q_shaft_TLU=[.125, .25, .5, 1, 1.5, 2] * 1e-3 m^3/s  p_diff_shaft_TLU=[.1, 1, 2] MPa  torque_shaft_TLU=[.47, 4.72, 9.35; .47, 4.7, 9.36; .47, 4.7, 9.4; .47, 4.7, 9.41; .47, 4.7, 9.46; .47, 4.68, 9.5] N*m  omega_shaft_TLU=[205, 80, 35; 455, 330, 285; 955, 831, 780; 1950, 1830, 1780; 2940, 2775, 2680; 3940, 3780, 3640] rpm  vol_eff_min=1e-3  vol_eff_max=1  mech_eff_min=1e-3  mech_eff_max=1  pressure_threshold=1e-3 MPa  omega_threshold=10 rad/s  supplied_range_check=simscape.enum.assert.action.none  motor_mode_check=simscape.enum.assert.action.none  pressure_check=simscape.enum.assert.action.none  p_min_valid=0.101325 MPa
      settings: InternalSimscapePortConfiguration="{\"Bottom\":[{\"id\":\"B\",\"label\":\"B\",\"type\":\"foundation.isothermal_liquid.isothermal_liquid\"}],\"Left\":[],\"Right\":[{\"id\":\"R\",\"label\":\"R\",\"type\":\"foundation.mechanical.rotational.rotational\"},{\"id\":\"C\",\"label\":\"C\",\"type\":\"foundation.mechanical.rotational.rotational\"}],\"Top\":[{\"id\":\"A\",\"label\":\"A\",\"type\":\"foundation.isothermal_liquid.isothermal_liquid\"}]}"
  S : Subsystem
      settings: PortSchema="{\"entries\":[{\"content\":{\"sides\":[{\"content\":{\"connectorIds\":[\"LConn1\"]},\"type\":\"ConnectorPlacement.EquallySpacedRectSide\",\"uuid\":\"d71b6971-6f33-4ff5-9472-1e7ceb29be5c\"},{\"content\":{\"connectorIds\":[\"Out1\",\"RConn1\"],\"side\":\"RIGHT\"},\"type\":\"ConnectorPlacement.EquallySpacedRectSide\",\"uuid\":\"20efd35b-04f1-44a0-a5ae-b6ecc8cce91a\"},{\"content\":{\"connectorIds\":[\"Out2\"],\"side\":\"TOP\"},\"type\":\"ConnectorPlacement.EquallySpacedRectSide\",\"uuid\":\"941ffbf3-e51b-4589-ab00-835957186b5f\"}]},\"type\":\"ConnectorPlacement.EquallySpacedConnector\",\"uuid\":\"7b30b026-434b-4245-94a4-5fd456974538\"}],\"packageUris\":[\"http://schema.mathworks.com/mf0/Connector/R2020b\"],\"version\":\"1.0\"}"
      mask Display: disp('S')
  A : PMIOPort  Side=Left
  R : PMIOPort  Port=2  Side=Right
  B : PMIOPort  Port=3  Side=Right
  Bus Element Out14 : Outport  PortName=m  Element=w (rpm)
  Bus Element Out1 : Outport  PortName=m  Element=trq (N*m)
  Bus Element Out2 : Outport  PortName=m  Element=q (m^3/s)
  wires:
  S/1(T (N*m)) -> Bus Element Out1/1
  S/2(w (rpm)) -> Bus Element Out14/1
  Q5/1(Q) -> Bus Element Out2/1
  connections:
  R/RConn1 -- S/RConn1
  Rear Axle Motor/RConn3 -- B/RConn1
  Q5/LConn1 -- Rear Axle Motor/LConn1
  Q5/RConn1 -- A/RConn1
  Rear Axle Motor/RConn2 -- Mechanical Rotational Reference/LConn1
  S/LConn1 -- Rear Axle Motor/RConn1

== system HydrostaticCVT/Relief Valve A ==
  Pressure Relief Valve A : SimscapeFluids_lib/Isothermal Liquid/Valves & Orifices/Pressure Control Valves/Pressure Relief Valve (IL)  set_pressure_spec=foundation.enum.constant_controlled.constant  opening_spec=fluids.isothermal_liquid.valves_orifices.enum.opening_spec.linear  pressure_spec=fluids.isothermal_liquid.valves_orifices.enum.pressure_control_spec.dp  p_set_gauge=0.1 MPa  p_set_differential=hydrostaticCVT.pressDifferentialSet MPa  p_range=hydrostaticCVT.pressRegulationRange MPa  area_max=hydrostaticCVT.maxArea m^2  area_leak=hydrostaticCVT.areaLeak m^2  p_diff_TLU=[0.2 : 0.2 : 1.2] MPa  p_gauge_TLU=[0.2 : 0.2 : 1.2] MPa  valve_area_TLU=[1e-10, 2e-06, 4e-06, 6e-06, 8e-06, 1e-05] m^2  vol_flow_TLU=[1e-09, 3.6e-05, 8.9e-05, .00015, .00023, .00031] m^3/s  area=inf m^2  Cd=hydrostaticCVT.cd  Re_c=150  smoothing_factor=0.01  pressure_recovery=simscape.enum.onoff.off  opening_dynamics=simscape.enum.onoff.off  tau=0.1 s
      settings: InternalSimscapePortConfiguration="{\"Bottom\":[],\"Left\":[{\"id\":\"A\",\"label\":\"A\",\"type\":\"foundation.isothermal_liquid.isothermal_liquid\"}],\"Right\":[{\"id\":\"B\",\"label\":\"B\",\"type\":\"foundation.isothermal_liquid.isothermal_liquid\"}],\"Top\":[]}"
  Q8 : Subsystem
      mask Display: disp('Q')
  A : PMIOPort  Side=Left
  B : PMIOPort  Port=2  Side=Right
  Bus Element Out12 : Outport  PortName=m  Element=q (m^3/s)
  wires:
  Q8/1(Q) -> Bus Element Out12/1
  connections:
  Pressure Relief Valve A/RConn1 -- B/RConn1
  Q8/LConn1 -- A/RConn1
  Q8/RConn1 -- Pressure Relief Valve A/LConn1

== system HydrostaticCVT/Relief Valve B ==
  Pressure Relief Valve B (bar) : SimscapeFluids_lib/Isothermal Liquid/Valves & Orifices/Pressure Control Valves/Pressure Relief Valve (IL)  set_pressure_spec=foundation.enum.constant_controlled.constant  opening_spec=fluids.isothermal_liquid.valves_orifices.enum.opening_spec.linear  pressure_spec=fluids.isothermal_liquid.valves_orifices.enum.pressure_control_spec.dp  p_set_gauge=0.1 MPa  p_set_differential=hydrostaticCVT.pressDifferentialSet MPa  p_range=hydrostaticCVT.pressRegulationRange MPa  area_max=hydrostaticCVT.maxArea m^2  area_leak=hydrostaticCVT.areaLeak m^2  p_diff_TLU=[0.2 : 0.2 : 1.2] MPa  p_gauge_TLU=[0.2 : 0.2 : 1.2] MPa  valve_area_TLU=[1e-10, 2e-06, 4e-06, 6e-06, 8e-06, 1e-05] m^2  vol_flow_TLU=[1e-09, 3.6e-05, 8.9e-05, .00015, .00023, .00031] m^3/s  area=inf m^2  Cd=hydrostaticCVT.cd  Re_c=150  smoothing_factor=0.01  pressure_recovery=simscape.enum.onoff.off  opening_dynamics=simscape.enum.onoff.off  tau=0.1 s
      settings: InternalSimscapePortConfiguration="{\"Bottom\":[],\"Left\":[{\"id\":\"A\",\"label\":\"A\",\"type\":\"foundation.isothermal_liquid.isothermal_liquid\"}],\"Right\":[{\"id\":\"B\",\"label\":\"B\",\"type\":\"foundation.isothermal_liquid.isothermal_liquid\"}],\"Top\":[]}"
  Q4 : Subsystem
      settings: PortSchema="{\"entries\":[{\"content\":{\"sides\":[{\"content\":{\"connectorIds\":[\"LConn1\"]},\"type\":\"ConnectorPlacement.EquallySpacedRectSide\",\"uuid\":\"a381c46d-7477-4f99-8d1a-7d1a868f6356\"},{\"content\":{\"connectorIds\":[\"RConn1\"],\"side\":\"RIGHT\"},\"type\":\"ConnectorPlacement.EquallySpacedRectSide\",\"uuid\":\"1773284f-5c53-4cb3-9146-19bcc89e0bf2\"},{\"content\":{\"side\":\"TOP\"},\"type\":\"ConnectorPlacement.EquallySpacedRectSide\",\"uuid\":\"2cc97cf0-3f11-430a-9e32-d4b384bcc7e2\"},{\"content\":{\"connectorIds\":[\"Out1\"],\"side\":\"BOTTOM\"},\"type\":\"ConnectorPlacement.EquallySpacedRectSide\",\"uuid\":\"c9ca2d64-d8c8-403a-a57b-d8b0d2fddcea\"}]},\"type\":\"ConnectorPlacement.EquallySpacedConnector\",\"uuid\":\"a3df120c-9f95-4600-8cbc-77d57dad487f\"}],\"packageUris\":[\"http://schema.mathworks.com/mf0/Connector/R2020b\"],\"version\":\"1.0\"}"
      mask Display: disp('Q')
  A : PMIOPort  Side=Left
  B : PMIOPort  Port=2  Side=Right
  Bus Element Out13 : Outport  PortName=m  Element=q (m^3/s)
  wires:
  Q4/1(Q) -> Bus Element Out13/1
  connections:
  Pressure Relief Valve B (bar)/RConn1 -- B/RConn1
  Q4/LConn1 -- A/RConn1
  Q4/RConn1 -- Pressure Relief Valve B (bar)/LConn1

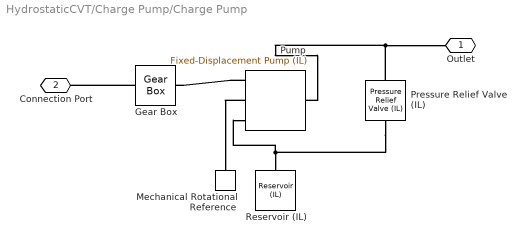
== system HydrostaticCVT/Charge Pump/Charge Pump ==
  Gear Box : fl_lib/Mechanical/Mechanisms/Gear Box  ratio=hydrostaticCVT.gearRatioAux  t_in_specify=off  t_in_priority=None  t_in=0 N*m  t_in_nominal_specify=off  t_in_nominal_value=1  t_in_nominal_unit=N*m  t_out_specify=off  t_out_priority=None  t_out=0 N*m  t_out_nominal_specify=off  t_out_nominal_value=1  t_out_nominal_unit=N*m
  Mechanical Rotational Reference : fl_lib/Mechanical/Rotational Elements/Mechanical Rotational Reference
  Pressure Relief Valve (IL) : SimscapeFluids_lib/Isothermal Liquid/Valves & Orifices/Pressure Control Valves/Pressure Relief Valve (IL)  set_pressure_spec=foundation.enum.constant_controlled.constant  opening_spec=fluids.isothermal_liquid.valves_orifices.enum.opening_spec.linear  pressure_spec=fluids.isothermal_liquid.valves_orifices.enum.pressure_control_spec.dp  p_set_gauge=0.1 MPa  p_set_differential=hydrostaticCVT.pressDifferentialSetAux MPa  p_range=hydrostaticCVT.pressRegulationRangeAux MPa  area_max=hydrostaticCVT.maxArea m^2  area_leak=hydrostaticCVT.areaLeak m^2  p_diff_TLU=[0.2 : 0.2 : 1.2] MPa  p_gauge_TLU=[0.2 : 0.2 : 1.2] MPa  valve_area_TLU=[1e-10, 2e-06, 4e-06, 6e-06, 8e-06, 1e-05] m^2  vol_flow_TLU=[1e-09, 3.6e-05, 8.9e-05, .00015, .00023, .00031] m^3/s  area=inf m^2  Cd=hydrostaticCVT.cd  Re_c=150  smoothing_factor=0.01  pressure_recovery=simscape.enum.onoff.off  opening_dynamics=simscape.enum.onoff.off  tau=0.1 s
      settings: InternalSimscapePortConfiguration="{\"Bottom\":[],\"Left\":[{\"id\":\"A\",\"label\":\"A\",\"type\":\"foundation.isothermal_liquid.isothermal_liquid\"}],\"Right\":[{\"id\":\"B\",\"label\":\"B\",\"type\":\"foundation.isothermal_liquid.isothermal_liquid\"}],\"Top\":[]}"
  Pump : SimscapeFluids_lib/Isothermal Liquid/Pumps & Motors/Fixed-Displacement Pump (IL)  leakage_friction_spec=fluids.isothermal_liquid.pumps_motors.enum.pump_motor_loss_spec.analytical  displacement=hydrostaticCVT.displacementPumpAux cm^3/rev  omega_nominal=hydrostaticCVT.shaftVelocityNominalAux rpm  p_nominal=hydrostaticCVT.nominalPressureGain MPa  vol_eff_nominal=hydrostaticCVT.efficiencyVolumetric  mech_eff_nominal=hydrostaticCVT.efficiencyMechanical  no_load_torque=0 N*m  p_diff_eff_TLU=[.1, 1, 2] MPa  omega_eff_TLU=[25, 50, 100, 200, 300, 400] rad/s  vol_eff_TLU=[.816, .908, .954, .977, .981, .984; .325, .663, .831, .916, .925, .946; .137, .568, .78, .892, .893, .91]  mech_eff_TLU=[.996, .996, .996, .996, .996, .996; .988, .989, .989, .989, .989, .99; .981, .981, .982, .982, .983, .984]  p_diff_loss_TLU=[.1, 1, 2] MPa  omega_loss_TLU=[25, 50, 100, 200, 300, 400] rad/s  vol_loss_TLU=[.023, .023, .023, .023, .0285, .032; .0844, .0842, .0845, .084, .1125, .108; .1079, .108, .11, .108, .1605, .18] * 1e-3 m^3/s  mech_loss_TLU=[.002, .002, .002, .002, .002, .002; .0607, .0556, .0556, .0556, .0556, .0505; .1937, .1937, .1833, .1833, .1729, .1626] N*m  vol_eff_min=1e-3  vol_eff_max=1  mech_eff_min=1e-3  mech_eff_max=1  pressure_threshold=1e-3 MPa  omega_threshold=10 rad/s  supplied_range_check=simscape.enum.assert.action.none  pump_mode_check=simscape.enum.assert.action.none  pressure_check=simscape.enum.assert.action.none  p_min_valid=0.101325 MPa
      settings: InternalSimscapePortConfiguration="{\"Bottom\":[{\"id\":\"A\",\"label\":\"A\",\"type\":\"foundation.isothermal_liquid.isothermal_liquid\"}],\"Left\":[],\"Right\":[{\"id\":\"R\",\"label\":\"R\",\"type\":\"foundation.mechanical.rotational.rotational\"},{\"id\":\"C\",\"label\":\"C\",\"type\":\"foundation.mechanical.rotational.rotational\"}],\"Top\":[{\"id\":\"B\",\"label\":\"B\",\"type\":\"foundation.isothermal_liquid.isothermal_liquid\"}]}"
  Reservoir (IL) : fl_lib/Isothermal Liquid/Elements/Reservoir (IL)  reservoir_type=foundation.enum.constant_controlled.constant  pressure_spec=foundation.enum.pressure_spec.atmospheric  reservoir_pressure=0.101325 MPa
  Outlet : PMIOPort  Side=Right
  Connection Port : PMIOPort  Port=2  Side=Left
  connections:
  Gear Box/LConn1 -- Connection Port/RConn1
  Pump/RConn1 -- Gear Box/RConn1
  Pump/RConn2 -- Mechanical Rotational Reference/LConn1
  Pump/RConn3 -- Pressure Relief Valve (IL)/RConn1 -- Reservoir (IL)/LConn1
  Pump/LConn1 -- Pressure Relief Valve (IL)/LConn1 -- Outlet/RConn1

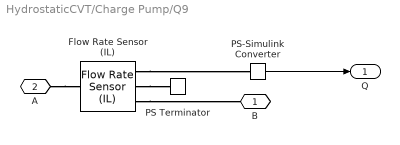
== system HydrostaticCVT/Charge Pump/Q9 ==
  Flow Rate Sensor (IL) : fl_lib/Isothermal Liquid/Sensors/Flow Rate Sensor (IL)  sensor_type=foundation.enum.mass_volumetric_sensor.mass_volumetric
      settings: InternalSimscapePortConfiguration="{\"Bottom\":[],\"Left\":[{\"id\":\"A\",\"label\":\"A\",\"type\":\"foundation.isothermal_liquid.isothermal_liquid\"}],\"Right\":[{\"id\":\"B\",\"label\":\"B\",\"type\":\"foundation.isothermal_liquid.isothermal_liquid\"},{\"id\":\"M\",\"label\":\"M\",\"type\":\"output\"},{\"id\":\"V\",\"label\":\"V\",\"type\":\"output\"}],\"Top\":[]}"
  PS Terminator : fl_lib/Physical Signals/Sinks/PS Terminator
  PS-Simulink Converter : nesl_utility/PS-Simulink Converter  PhysicalDomain=network_engine_domain  SubClassName=ps_output  LeftPortType=input  RightPortType=output  PseudoPeriodic=off  Frequencies=[]  VectorFormat=1-D array  Unit=m^3/s  AffineConversion=off
  B : PMIOPort  Side=Left
  A : PMIOPort  Port=2  Side=Right
  Q : Outport
  wires:
  PS-Simulink Converter/1 -> Q/1
  connections:
  A/RConn1 -- Flow Rate Sensor (IL)/LConn1
  Flow Rate Sensor (IL)/RConn1 -- B/RConn1
  Flow Rate Sensor (IL)/RConn3 -- PS-Simulink Converter/LConn1
  Flow Rate Sensor (IL)/RConn2 -- PS Terminator/LConn1

== system HydrostaticCVT/Charge Pump/T1 ==
  PS2S : nesl_utility/PS-Simulink Converter  PhysicalDomain=network_engine_domain  SubClassName=ps_output  LeftPortType=input  RightPortType=output  PseudoPeriodic=off  Frequencies=[]  VectorFormat=1-D array  Unit=N*m  AffineConversion=off
  Torque Sensor : fl_lib/Mechanical/Mechanical Sensors/Ideal Torque Sensor
  A : PMIOPort  Side=Left
  B : PMIOPort  Port=2  Side=Right
  T : Outport
  wires:
  PS2S/1 -> T/1
  connections:
  B/RConn1 -- Torque Sensor/RConn1
  Torque Sensor/RConn2 -- PS2S/LConn1
  A/RConn1 -- Torque Sensor/LConn1

== system HydrostaticCVT/Charge Pump/p4 ==
  PS-Simulink Converter : nesl_utility/PS-Simulink Converter  PhysicalDomain=network_engine_domain  SubClassName=ps_output  LeftPortType=input  RightPortType=output  PseudoPeriodic=off  Frequencies=[]  VectorFormat=1-D array  Unit=bar  AffineConversion=off
  Pressure Sensor (IL) : fl_lib/Isothermal Liquid/Sensors/Pressure Sensor (IL)  pressure_measure=foundation.enum.pressure_measure.difference
      settings: InternalSimscapePortConfiguration="{\"Bottom\":[],\"Left\":[{\"id\":\"A\",\"label\":\"A\",\"type\":\"foundation.isothermal_liquid.isothermal_liquid\"}],\"Right\":[{\"id\":\"B\",\"label\":\"B\",\"type\":\"foundation.isothermal_liquid.isothermal_liquid\"},{\"id\":\"P\",\"label\":\"P\",\"type\":\"output\"}],\"Top\":[]}"
  Reservoir (IL)1 : fl_lib/Isothermal Liquid/Elements/Reservoir (IL)  reservoir_type=foundation.enum.constant_controlled.constant  pressure_spec=foundation.enum.pressure_spec.atmospheric  reservoir_pressure=0.101325 MPa
  A : PMIOPort  Side=Left
  " P" : Outport
  wires:
  PS-Simulink Converter/1 -> " P"/1
  connections:
  Pressure Sensor (IL)/LConn1 -- A/RConn1
  Reservoir (IL)1/LConn1 -- Pressure Sensor (IL)/RConn1
  PS-Simulink Converter/LConn1 -- Pressure Sensor (IL)/RConn2

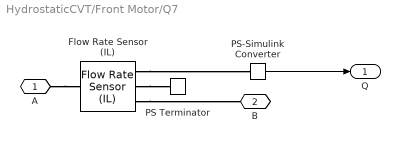
== system HydrostaticCVT/Front Motor/Q7 ==
  Flow Rate Sensor (IL) : fl_lib/Isothermal Liquid/Sensors/Flow Rate Sensor (IL)  sensor_type=foundation.enum.mass_volumetric_sensor.mass_volumetric
      settings: InternalSimscapePortConfiguration="{\"Bottom\":[],\"Left\":[{\"id\":\"A\",\"label\":\"A\",\"type\":\"foundation.isothermal_liquid.isothermal_liquid\"}],\"Right\":[{\"id\":\"B\",\"label\":\"B\",\"type\":\"foundation.isothermal_liquid.isothermal_liquid\"},{\"id\":\"M\",\"label\":\"M\",\"type\":\"output\"},{\"id\":\"V\",\"label\":\"V\",\"type\":\"output\"}],\"Top\":[]}"
  PS Terminator : fl_lib/Physical Signals/Sinks/PS Terminator
  PS-Simulink Converter : nesl_utility/PS-Simulink Converter  PhysicalDomain=network_engine_domain  SubClassName=ps_output  LeftPortType=input  RightPortType=output  PseudoPeriodic=off  Frequencies=[]  VectorFormat=1-D array  Unit=m^3/s  AffineConversion=off
  A : PMIOPort  Side=Left
  B : PMIOPort  Port=2  Side=Right
  Q : Outport
  wires:
  PS-Simulink Converter/1 -> Q/1
  connections:
  Flow Rate Sensor (IL)/RConn2 -- PS Terminator/LConn1
  Flow Rate Sensor (IL)/RConn3 -- PS-Simulink Converter/LConn1
  Flow Rate Sensor (IL)/RConn1 -- B/RConn1
  A/RConn1 -- Flow Rate Sensor (IL)/LConn1

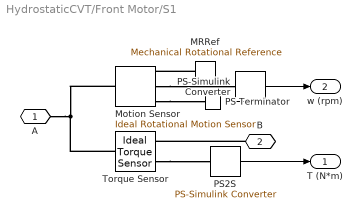
== system HydrostaticCVT/Front Motor/S1 ==
  MRRef : fl_lib/Mechanical/Rotational Elements/Mechanical Rotational Reference
  Motion Sensor : fl_lib/Mechanical/Mechanical Sensors/Ideal Rotational Motion Sensor  reference=foundation.enum.MeasurementReference.difference  acceleration_port=false  velocity_port=true  position_port=true  wrap_angle=simscape.enum.onoff.off  offset=0 rad
  PS Terminator : fl_lib/Physical Signals/Sinks/PS Terminator
  PS-Simulink Converter : nesl_utility/PS-Simulink Converter  PhysicalDomain=network_engine_domain  SubClassName=ps_output  LeftPortType=input  RightPortType=output  PseudoPeriodic=off  Frequencies=[]  VectorFormat=1-D array  Unit=rpm  AffineConversion=off
  PS2S : nesl_utility/PS-Simulink Converter  PhysicalDomain=network_engine_domain  SubClassName=ps_output  LeftPortType=input  RightPortType=output  PseudoPeriodic=off  Frequencies=[]  VectorFormat=1-D array  Unit=N*m  AffineConversion=off
  Torque Sensor : fl_lib/Mechanical/Mechanical Sensors/Ideal Torque Sensor
  A : PMIOPort  Side=Left
  B : PMIOPort  Port=2  Side=Right
  T (N*m) : Outport
  w (rpm) : Outport  Port=2
  wires:
  PS2S/1 -> T (N*m)/1
  PS-Simulink Converter/1 -> w (rpm)/1
  connections:
  Torque Sensor/LConn1 -- A/RConn1 -- Motion Sensor/LConn1
  Motion Sensor/RConn2 -- PS-Simulink Converter/LConn1
  MRRef/LConn1 -- Motion Sensor/RConn1
  Torque Sensor/RConn2 -- PS2S/LConn1
  B/RConn1 -- Torque Sensor/RConn1
  Motion Sensor/RConn3 -- PS Terminator/LConn1

== system HydrostaticCVT/Main Pump/Q11 ==
  Flow Rate Sensor (IL) : fl_lib/Isothermal Liquid/Sensors/Flow Rate Sensor (IL)  sensor_type=foundation.enum.mass_volumetric_sensor.mass_volumetric
      settings: InternalSimscapePortConfiguration="{\"Bottom\":[],\"Left\":[{\"id\":\"A\",\"label\":\"A\",\"type\":\"foundation.isothermal_liquid.isothermal_liquid\"}],\"Right\":[{\"id\":\"B\",\"label\":\"B\",\"type\":\"foundation.isothermal_liquid.isothermal_liquid\"},{\"id\":\"M\",\"label\":\"M\",\"type\":\"output\"},{\"id\":\"V\",\"label\":\"V\",\"type\":\"output\"}],\"Top\":[]}"
  PS Terminator : fl_lib/Physical Signals/Sinks/PS Terminator
  PS-Simulink Converter : nesl_utility/PS-Simulink Converter  PhysicalDomain=network_engine_domain  SubClassName=ps_output  LeftPortType=input  RightPortType=output  PseudoPeriodic=off  Frequencies=[]  VectorFormat=1-D array  Unit=m^3/s  AffineConversion=off
  A : PMIOPort  Side=Left
  B : PMIOPort  Port=2  Side=Right
  Q : Outport
  wires:
  PS-Simulink Converter/1 -> Q/1
  connections:
  A/RConn1 -- Flow Rate Sensor (IL)/LConn1
  Flow Rate Sensor (IL)/RConn1 -- B/RConn1
  Flow Rate Sensor (IL)/RConn3 -- PS-Simulink Converter/LConn1
  Flow Rate Sensor (IL)/RConn2 -- PS Terminator/LConn1

== system HydrostaticCVT/Main Pump/T2 ==
  PS2S : nesl_utility/PS-Simulink Converter  PhysicalDomain=network_engine_domain  SubClassName=ps_output  LeftPortType=input  RightPortType=output  PseudoPeriodic=off  Frequencies=[]  VectorFormat=1-D array  Unit=N*m  AffineConversion=off
  Torque Sensor : fl_lib/Mechanical/Mechanical Sensors/Ideal Torque Sensor
  A : PMIOPort  Side=Left
  B : PMIOPort  Port=2  Side=Right
  T : Outport
  wires:
  PS2S/1 -> T/1
  connections:
  A/RConn1 -- Torque Sensor/LConn1
  Torque Sensor/RConn2 -- PS2S/LConn1
  B/RConn1 -- Torque Sensor/RConn1

== system HydrostaticCVT/Pipe A/Q10 ==
  Flow Rate Sensor (IL) : fl_lib/Isothermal Liquid/Sensors/Flow Rate Sensor (IL)  sensor_type=foundation.enum.mass_volumetric_sensor.mass_volumetric
      settings: InternalSimscapePortConfiguration="{\"Bottom\":[],\"Left\":[{\"id\":\"A\",\"label\":\"A\",\"type\":\"foundation.isothermal_liquid.isothermal_liquid\"}],\"Right\":[{\"id\":\"B\",\"label\":\"B\",\"type\":\"foundation.isothermal_liquid.isothermal_liquid\"},{\"id\":\"M\",\"label\":\"M\",\"type\":\"output\"},{\"id\":\"V\",\"label\":\"V\",\"type\":\"output\"}],\"Top\":[]}"
  PS Terminator : fl_lib/Physical Signals/Sinks/PS Terminator
  PS-Simulink Converter : nesl_utility/PS-Simulink Converter  PhysicalDomain=network_engine_domain  SubClassName=ps_output  LeftPortType=input  RightPortType=output  PseudoPeriodic=off  Frequencies=[]  VectorFormat=1-D array  Unit=m^3/s  AffineConversion=off
  A : PMIOPort  Side=Left
  B : PMIOPort  Port=2  Side=Right
  Q : Outport
  wires:
  PS-Simulink Converter/1 -> Q/1
  connections:
  A/RConn1 -- Flow Rate Sensor (IL)/LConn1
  Flow Rate Sensor (IL)/RConn1 -- B/RConn1
  Flow Rate Sensor (IL)/RConn3 -- PS-Simulink Converter/LConn1
  Flow Rate Sensor (IL)/RConn2 -- PS Terminator/LConn1

== system HydrostaticCVT/Pipe A/Q2 ==
  Flow Rate Sensor (IL) : fl_lib/Isothermal Liquid/Sensors/Flow Rate Sensor (IL)  sensor_type=foundation.enum.mass_volumetric_sensor.mass_volumetric
      settings: InternalSimscapePortConfiguration="{\"Bottom\":[],\"Left\":[{\"id\":\"A\",\"label\":\"A\",\"type\":\"foundation.isothermal_liquid.isothermal_liquid\"}],\"Right\":[{\"id\":\"B\",\"label\":\"B\",\"type\":\"foundation.isothermal_liquid.isothermal_liquid\"},{\"id\":\"M\",\"label\":\"M\",\"type\":\"output\"},{\"id\":\"V\",\"label\":\"V\",\"type\":\"output\"}],\"Top\":[]}"
  PS Terminator : fl_lib/Physical Signals/Sinks/PS Terminator
  PS-Simulink Converter : nesl_utility/PS-Simulink Converter  PhysicalDomain=network_engine_domain  SubClassName=ps_output  LeftPortType=input  RightPortType=output  PseudoPeriodic=off  Frequencies=[]  VectorFormat=1-D array  Unit=m^3/s  AffineConversion=off
  A : PMIOPort  Side=Left
  B : PMIOPort  Port=2  Side=Right
  Q : Outport
  wires:
  PS-Simulink Converter/1 -> Q/1
  connections:
  Flow Rate Sensor (IL)/RConn2 -- PS Terminator/LConn1
  Flow Rate Sensor (IL)/RConn3 -- PS-Simulink Converter/LConn1
  Flow Rate Sensor (IL)/RConn1 -- B/RConn1
  A/RConn1 -- Flow Rate Sensor (IL)/LConn1
